simulink model "TempControl_OpenLoop_sakai_2026a"  (R2026b)
settings: Solver=FixedStepDiscrete  StopTime=600  FixedStep=10e-3  EnableMultiTasking=on
libraries: mbedblockslib x2
settings Model: SILPILModeSetting=veronly  Creator=Lukas  LastModifiedBy=ursmu
settings OptimizationCC: DifferentSizesBufferReuse=on  EnhancedBackFolding=on  MaxStackSize=64  OptimizationCustomize=off  OptimizeBlockOrder=speed
settings DebuggingCC: ParameterTunabilityLossMsg=error
settings HardwareCC: ProdHWDeviceType=ARM Compatible->ARM Cortex  ProdLargestAtomicFloat=Double  ProdLargestAtomicInteger=Long  ProdLongLongMode=on
settings SFSimCC: MATLABDynamicMemAlloc=off
settings RTWCC: Description=Embedded Coder  HardwareBoard=STM32 Nucleo F401RE  SystemTargetFile=ert.tlc  TLCOptions=-aInlineSetEventsForThisBaseRateFcn=TLC_FALSE -aSuppressMultiTaskScheduler=TLC_FALSE -aRateBasedStepFcn=1  TemplateMakefile=ert_default_tmf  Toolchain=GNU Tools for STM32
settings CodeAppCC: ForceParamTrailComments=on  OperatorAnnotations=on
settings ERTTargetCC: CodeReplacementLibrary=ARM Cortex-M  DynamicArrayContainerType=coder::array  ERTCustomFileBanners=off  ExtModeIntrfLevel=Level2 - Open  ExtModeMexFile=ext_xcp  ExtModeStaticAlloc=on  ModelStepFunctionPrototypeControlCompliant=off  SupportContinuousTime=on  SupportNonInlinedSFcns=on

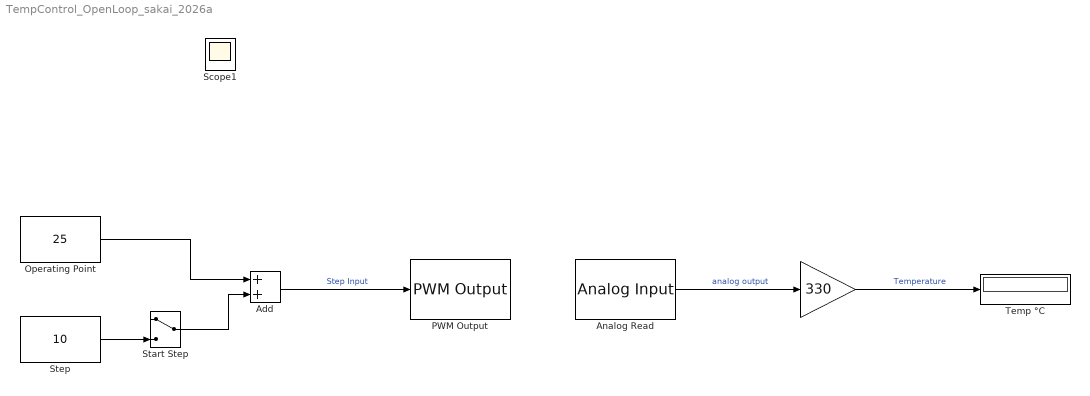
== system TempControl_OpenLoop_sakai_2026a ==
  " " : Gain  Gain=330
  Add : Sum
  Analog Read : mbedblockslib/Analog Input  Pin=A0  ReadResultsOnly=off  ConversionTriggerSource=Software  ExternalTriggerType=uint32( 0 )  OutputDataType=double  EnableConversionCompleteNotify=off  EnableOuputStatus=off  SampleTime=10e-3
      settings: LibrarySourceBlock=stmnucleorootlib/Common/Analog Input
  Operating Point : Constant  Value=25  SampleTime=10e-3
  PWM Output : mbedblockslib/PWM Output  Pin=D2  EnableInputFrequency=off  InitialFrequency=10000  InitialDutyCycle=20  NotificationType=None
      settings: LibrarySourceBlock=stmnucleorootlib/Common/PWM Output
  Start Step : ManualSwitch
  Step : Constant  Value=10  SampleTime=10e-3
  Temp °C : Display
  Scope1 : Scope
      settings: ActiveDisplayYMinimum=20.9423  ActiveDisplayYMaximum=22.6548
  wires:
  Operating Point/1 -> Add/1
  Add/1 -> PWM Output/1  "Step Input"
  Step/1 -> Start Step/2
  Start Step/1 -> Add/2
  Analog Read/1 -> " "/1  "analog output"
  " "/1 -> Temp °C/1  "Temperature"
